simulink model "Prado23210715YP4"  (R2023a)
settings: Solver=VariableStepAuto  StartTime=0.0  StopTime=10.0  MaxStep=1E-3  RelTol=1e-3
libraries: fl_lib x14, nesl_utility x6, slpidlib x1
settings Model: Creator=adrib  LastModifiedBy=IT
settings DataIOCC: SaveFormat=Array  ReturnWorkspaceOutputs=off  TimeSaveName=t
settings DebuggingCC: AlgebraicLoopMsg=none  ArtificialAlgebraicLoopMsg=none  MaxConsecutiveZCsMsg=none  ModelReferenceExtraNoncontSigs=none  OperatingPointInterfaceChecksumMismatchMsg=none

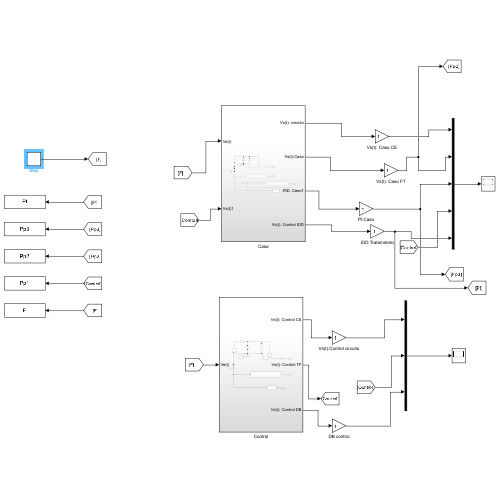
[thumbnail: Simulink's stored preview of the top-level diagram]
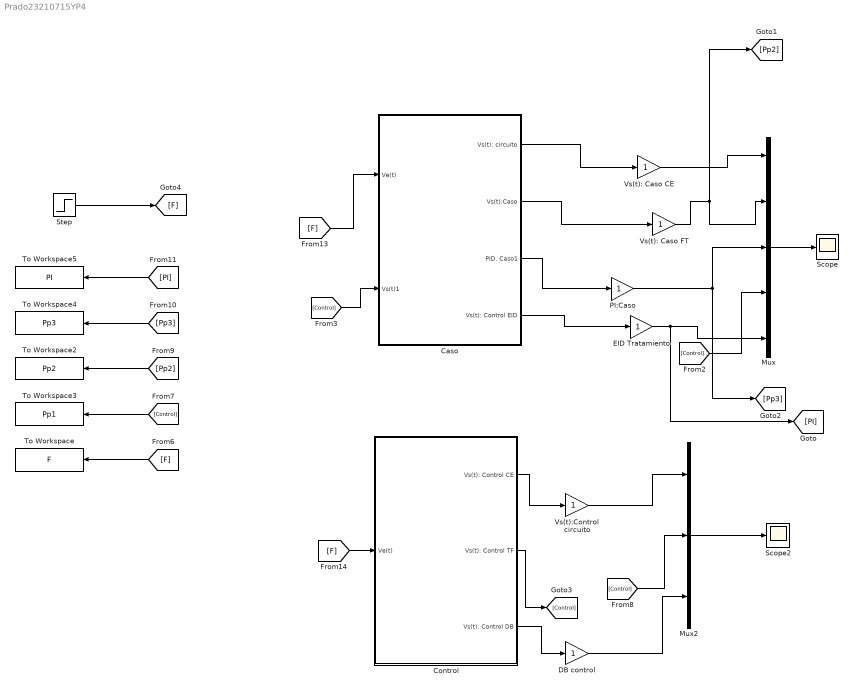
== system Prado23210715YP4 ==
  Caso : Subsystem
  Control : Subsystem
  DB control : Gain
  EID Tratamiento : Gain
  Mux : Mux  Inputs=5
  Mux2 : Mux  Inputs=3
  PI:Caso : Gain
  Scope : Scope
  Scope2 : Scope
  Step : Step  Time=0  SampleTime=0
  To Workspace : ToWorkspace  VariableName=F  SampleTime=-1
  To Workspace2 : ToWorkspace  VariableName=Pp2  SampleTime=-1
  To Workspace3 : ToWorkspace  VariableName=Pp1  SampleTime=-1
  To Workspace4 : ToWorkspace  VariableName=Pp3  SampleTime=-1
  To Workspace5 : ToWorkspace  VariableName=PI  SampleTime=-1
  Vs(t): Caso CE : Gain
  Vs(t): Caso FT : Gain
  Vs(t):Control circuito : Gain
  wires:
  Mux/1 -> Scope/1
  Mux2/1 -> Scope2/1
  [F] -> To Workspace/1
  [Control] -> To Workspace3/1
  [Pp2] -> To Workspace2/1
  [Pp3] -> To Workspace4/1
  [PI] -> To Workspace5/1
  [F] -> Control/1(Ve(t))
  Step/1 -> [F]
  Caso/1(Vs(t): circuito) -> Vs(t): Caso CE/1
  Vs(t): Caso FT/1 -> [Pp2], Mux/2
  [F] -> Caso/1(Ve(t))
  Caso/2(Vs(t):Caso) -> Vs(t): Caso FT/1
  Caso/3(PID. Caso1) -> PI:Caso/1
  [Control] -> Mux/4
  [Control] -> Caso/2(Vs(t)1)
  Control/2(Vs(t): Control TF) -> [Control]
  [Control] -> Mux2/2
  Control/1(Vs(t): Control CE) -> Vs(t):Control circuito/1
  Vs(t):Control circuito/1 -> Mux2/1
  Caso/4(Vs(t): Control EID) -> EID Tratamiento/1
  EID Tratamiento/1 -> [PI], Mux/5
  Control/3(Vs(t): Control DB) -> DB control/1
  DB control/1 -> Mux2/3
  Vs(t): Caso CE/1 -> Mux/1
  PI:Caso/1 -> [Pp3], Mux/3

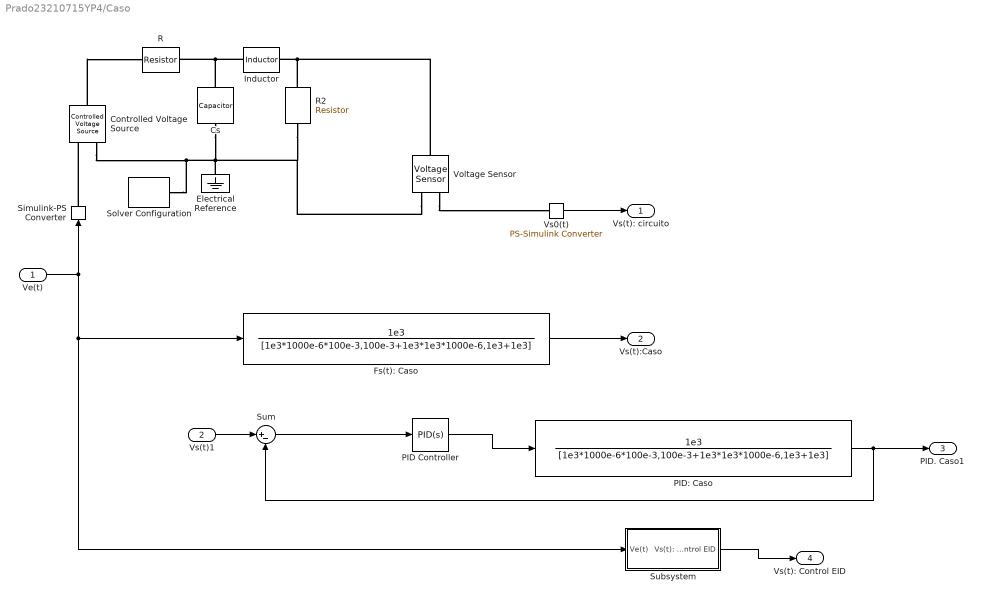
== system Prado23210715YP4/Caso ==
  Ve(t) : Inport
  Vs(t)1 : Inport  Port=2
  Controlled Voltage Source : fl_lib/Electrical/Electrical Sources/Controlled Voltage Source
  Cs : fl_lib/Electrical/Electrical Elements/Capacitor  c=1000e-6 F  r=1e-6 Ohm  g=0 1/Ohm  i_specify=off  i_priority=None  i=0 A  i_nominal_specify=off  i_nominal_unit=A  i_nominal_value=1  v_specify=off  v_priority=None  v=0 V  v_nominal_specify=off  v_nominal_unit=V  v_nominal_value=1  vc_specify=off  vc_priority=High  vc=0 V  vc_nominal_specify=off  vc_nominal_unit=V  vc_nominal_value=1
  Electrical Reference : fl_lib/Electrical/Electrical Elements/Electrical Reference
  Fs(t): Caso : TransferFcn  Numerator=[1e3]  Denominator=[1e3*1000e-6*100e-3,100e-3+1e3*1e3*1000e-6,1e3+1e3]
  Inductor : fl_lib/Electrical/Electrical Elements/Inductor  l=100e-3 H  r=0 Ohm  g=1e-9 1/Ohm  i_specify=off  i_priority=None  i=0 A  i_nominal_specify=off  i_nominal_unit=A  i_nominal_value=1  v_specify=off  v_priority=None  v=0 V  v_nominal_specify=off  v_nominal_unit=V  v_nominal_value=1  i_L_specify=off  i_L_priority=High  i_L=0 A  i_L_nominal_specify=off  i_L_nominal_unit=A  i_L_nominal_value=1
  PID Controller : slpidlib/PID Controller  Controller=PID  Form=Parallel  TimeDomain=Continuous-time  UseExternalTs=off  SampleTime=-1  IntegratorMethod=Forward Euler  FilterMethod=Forward Euler  ControllerParametersSource=internal  P=1315.6500509428  I=314901.771136491  UseKiTs=off  D=0.310353252867865  N=7592.76369465997  UseFilter=on  TunerSelectOption=Transfer Function Based (PID Tuner App)  InitialConditionSource=internal  InitialConditionForIntegrator=0  InitialConditionForFilter=0  DifferentiatorICPrevScaledInput=0  ExternalReset=none  TrackingMode=off  Kt=1  LimitOutput=off  SatLimitsSource=internal  UpperSaturationLimit=inf  LowerSaturationLimit=-inf  LinearizeAsGain=on  AntiWindupMode=none  Kb=1  LimitIntegrator=off  UpperIntegratorSaturationLimit=inf  LowerIntegratorSaturationLimit=-inf  POutMin=[]  POutMax=[]  IOutMin=[]  IOutMax=[]  DOutMin=[]  DOutMax=[]  NOutMin=[]  NOutMax=[]  SumOutMin=[]  SumOutMax=[]  SaturationOutMin=[]  SaturationOutMax=[]  PParamMin=[]  PParamMax=[]  IParamMin=[]  IParamMax=[]  DParamMin=[]  DParamMax=[]  NParamMin=[]  NParamMax=[]  KbParamMin=[]  KbParamMax=[]  KtParamMin=[]  KtParamMax=[]  KbOutMin=[]  KbOutMax=[]  KtOutMin=[]  KtOutMax=[]  IntegratorOutMin=[]  IntegratorOutMax=[]  FilterOutMin=[]  FilterOutMax=[]  SumI1OutMin=[]  SumI1OutMax=[]  SumI2OutMin=[]  SumI2OutMax=[]  SumI3OutMin=[]  SumI3OutMax=[]  SumI4OutMin=[]  SumI4OutMax=[]  SumDOutMin=[]  SumDOutMax=[]  DifferentiatorOutMin=[]  DifferentiatorOutMax=[]  FilterDiffOutCoefMin=[]  FilterDiffOutCoefMax=[]  ReciprocalOutMin=[]  ReciprocalOutMax=[]  SumDenOutMin=[]  SumDenOutMax=[]  SumNumOutMin=[]  SumNumOutMax=[]  DivideOutMin=[]  DivideOutMax=[]  UdiffTsProdOutMin=[]  UdiffTsProdOutMax=[]  NTsProdOutMin=[]  NTsProdOutMax=[]  UintegralTsProdOutMin=[]  UintegralTsProdOutMax=[]  UngainTsProdOutMin=[]  UngainTsProdOutMax=[]  ClampingZeroOutDataTypeStr=Inherit: Inherit via back propagation  ClampingZeroOutMin=[]  ClampingZeroOutMax=[]  FilterDenConstantOutDataTypeStr=Inherit: Inherit via back propagation  FilterDenConstantOutMin=[]  FilterDenConstantOutMax=[]  PCopyOutDataTypeStr=Inherit: Inherit via back propagation  PCopyOutMin=[]  PCopyOutMax=[]  NCopyOutDataTypeStr=Inherit: Inherit via back propagation  NCopyOutMin=[]  NCopyOutMax=[]  IntegratorContinuousStateAttributes=''  IntegratorStateMustResolveToSignalObject=off  IntegratorRTWStateStorageClass=Auto  FilterContinuousStateAttributes=''  FilterStateMustResolveToSignalObject=off  FilterRTWStateStorageClass=Auto  ParallelPVariant=InternalParameters  IdealPVariant=Disabled  IVariant=InternalParameters  DVariant=InternalParameters  IntegratorVariant=Continuous  SatVariant=Disabled  AWVariant=Passthrough  PCopyVariant=Disabled  TRVariant=Disabled  FdbkBlocksVariant=Forward  IdealPFdbkVariant=Disabled  SatFdbkVariant=Disabled  DerivativeFilterVariant=ContFilter  NVariant=InternalParameters  NCopyVariant=Disabled  FilterICVariant=InternalICsFilter  IntegratorICVariant=InternalICs  ExternalResetVariant=Disabled  TRSumVariant=Passthrough  SumFdbkVariant=Disabled  SumVariant=Sum_PID  TsampFilterVariant=InternalTs  TsampNgainVariant=Passthrough  TsampIntegralVariant=Disabled_SignalSpec  ExternalSaturationOutDataTypeStr=Inherit: Same as second input
  PID: Caso : TransferFcn  Numerator=[1e3]  Denominator=[1e3*1000e-6*100e-3,100e-3+1e3*1e3*1000e-6,1e3+1e3]
  R : fl_lib/Electrical/Electrical Elements/Resistor  R=1 kOhm  i_specify=off  i_priority=None  i=0 A  i_nominal_specify=off  i_nominal_unit=A  i_nominal_value=1  v_specify=off  v_priority=None  v=0 V  v_nominal_specify=off  v_nominal_unit=V  v_nominal_value=1
  R2 : fl_lib/Electrical/Electrical Elements/Resistor  R=1 kOhm  i_specify=off  i_priority=None  i=0 A  i_nominal_specify=off  i_nominal_unit=A  i_nominal_value=1  v_specify=off  v_priority=None  v=0 V  v_nominal_specify=off  v_nominal_unit=V  v_nominal_value=1
  Simulink-PS Converter : nesl_utility/Simulink-PS Converter  PhysicalDomain=network_engine_domain  SubClassName=ps_input  LeftPortType=input  RightPortType=output  PseudoPeriodic=off  Frequencies=[]  NoiseDistribution=none  NoiseParameters=[]  Unit=1  AffineConversion=off  FilteringAndDerivatives=provide  SimscapeFilterOrder=1  InputFilterTimeConstant=0.001  UdotUserProvided=0
  Solver Configuration : nesl_utility/Solver Configuration  PhysicalDomain=network_engine_domain  SubClassName=solver  LeftPortType=input  RightPortType=generic  Tones=[]  Harmonics=[]  SimulateNoise=off  Profile=off  UseLocalSampling=off  EnableSwitchedLinearOptims=on  FrequencyDomain=off  UseCCode=off  RelTol=0.001  AbsTol=0.001  MinStep=1e-09  ToWorkspace=off  RevertToSquareIcSolve=off  NumHomotopyIterations=100  PhasorMode=off  PhasorModeNumHarmonics=1  ConsistencySolver=NEWTON_XTOL_AFTER_FTOL  IndexReductionMethod=DerivativeReplacement  DoDC=off  ResidualTolerance=1e-09  ConsistencyTolSource=GLOBAL  ConsistencyAbsTol=0.001  ConsistencyRelTol=0.001  ConsistencyTolFactor=0.001  UseLocalSolver=off  LocalSolverChoice=NE_BACKWARD_EULER_ADVANCER  ResolveIndetEquations=on  FunctionEvalNumThread=1  LocalSolverSampleTime=0.001  DoFixedCost=off  MaxNonlinIter=3  MaxModeIter=2  ComputeImpulses=off  ImpulseIterations=2  LinearAlgebra=auto  LinearAlgebraNumThread=0  EquationFormulation=NE_TIME_EF  DelaysMemoryBudget=1024  AutomaticFiltering=on  FilteringTimeConstant=0.001  PartitionStorageMethod=AS_NEEDED  PartitionMemoryBudget=1024  PartitionMethod=ROBUST
  Subsystem : Subsystem
  Sum : Sum  Inputs=|+-
  Voltage Sensor : fl_lib/Electrical/Electrical Sensors/Voltage Sensor
  Vs0(t) : nesl_utility/PS-Simulink Converter  PhysicalDomain=network_engine_domain  SubClassName=ps_output  LeftPortType=input  RightPortType=output  PseudoPeriodic=off  Frequencies=[]  VectorFormat=1-D array  Unit=inherit  AffineConversion=off
  Vs(t): circuito : Outport
  Vs(t):Caso : Outport  Port=2
  PID. Caso1 : Outport  Port=3
  Vs(t): Control EID : Outport  Port=4
  wires:
  Fs(t): Caso/1 -> Vs(t):Caso/1
  Vs0(t)/1 -> Vs(t): circuito/1
  Ve(t)/1 -> Simulink-PS Converter/1, Subsystem/1(Ve(t)), Fs(t): Caso/1
  Sum/1 -> PID Controller/1
  PID: Caso/1 -> Sum/2, PID. Caso1/1
  PID Controller/1 -> PID: Caso/1
  Vs(t)1/1 -> Sum/1
  Subsystem/1(Vs(t): Control EID) -> Vs(t): Control EID/1
  connections:
  Controlled Voltage Source/RConn2 -- R2/LConn1 -- Voltage Sensor/RConn2 -- Cs/LConn1 -- Electrical Reference/LConn1 -- Solver Configuration/RConn1
  Voltage Sensor/RConn1 -- Vs0(t)/LConn1
  Simulink-PS Converter/RConn1 -- Controlled Voltage Source/RConn1
  Controlled Voltage Source/LConn1 -- R/RConn1
  Inductor/LConn1 -- Cs/RConn1 -- R/LConn1
  Voltage Sensor/LConn1 -- R2/RConn1 -- Inductor/RConn1

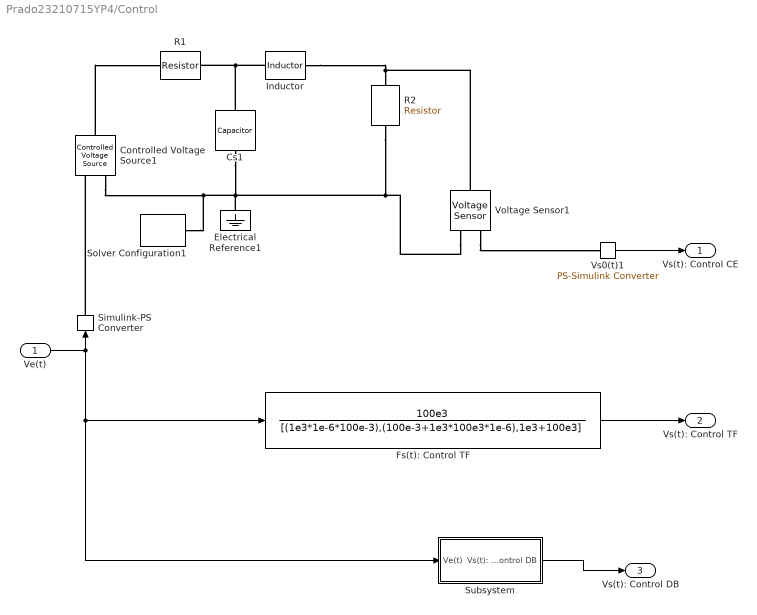
== system Prado23210715YP4/Control ==
  Ve(t) : Inport
  Controlled Voltage Source1 : fl_lib/Electrical/Electrical Sources/Controlled Voltage Source
  Cs1 : fl_lib/Electrical/Electrical Elements/Capacitor  c=1e-6 F  r=1e-6 Ohm  g=0 1/Ohm  i_specify=off  i_priority=None  i=0 A  i_nominal_specify=off  i_nominal_unit=A  i_nominal_value=1  v_specify=off  v_priority=None  v=0 V  v_nominal_specify=off  v_nominal_unit=V  v_nominal_value=1  vc_specify=off  vc_priority=High  vc=0 V  vc_nominal_specify=off  vc_nominal_unit=V  vc_nominal_value=1
  Electrical Reference1 : fl_lib/Electrical/Electrical Elements/Electrical Reference
  Fs(t): Control TF : TransferFcn  Numerator=[100e3]  Denominator=[(1e3*1e-6*100e-3),(100e-3+1e3*100e3*1e-6),1e3+100e3]
  Inductor : fl_lib/Electrical/Electrical Elements/Inductor  l=100e-3 H  r=0 Ohm  g=1e-9 1/Ohm  i_specify=off  i_priority=None  i=0 A  i_nominal_specify=off  i_nominal_unit=A  i_nominal_value=1  v_specify=off  v_priority=None  v=0 V  v_nominal_specify=off  v_nominal_unit=V  v_nominal_value=1  i_L_specify=off  i_L_priority=High  i_L=0 A  i_L_nominal_specify=off  i_L_nominal_unit=A  i_L_nominal_value=1
  R1 : fl_lib/Electrical/Electrical Elements/Resistor  R=1 kOhm  i_specify=off  i_priority=None  i=0 A  i_nominal_specify=off  i_nominal_unit=A  i_nominal_value=1  v_specify=off  v_priority=None  v=0 V  v_nominal_specify=off  v_nominal_unit=V  v_nominal_value=1
  R2 : fl_lib/Electrical/Electrical Elements/Resistor  R=100 kOhm  i_specify=off  i_priority=None  i=0 A  i_nominal_specify=off  i_nominal_unit=A  i_nominal_value=1  v_specify=off  v_priority=None  v=0 V  v_nominal_specify=off  v_nominal_unit=V  v_nominal_value=1
  Simulink-PS Converter : nesl_utility/Simulink-PS Converter  PhysicalDomain=network_engine_domain  SubClassName=ps_input  LeftPortType=input  RightPortType=output  PseudoPeriodic=off  Frequencies=[]  NoiseDistribution=none  NoiseParameters=[]  Unit=1  AffineConversion=off  FilteringAndDerivatives=provide  SimscapeFilterOrder=1  InputFilterTimeConstant=0.001  UdotUserProvided=0
  Solver Configuration1 : nesl_utility/Solver Configuration  PhysicalDomain=network_engine_domain  SubClassName=solver  LeftPortType=input  RightPortType=generic  Tones=[]  Harmonics=[]  SimulateNoise=off  Profile=off  UseLocalSampling=off  EnableSwitchedLinearOptims=on  FrequencyDomain=off  UseCCode=off  RelTol=0.001  AbsTol=0.001  MinStep=1e-09  ToWorkspace=off  RevertToSquareIcSolve=off  NumHomotopyIterations=100  PhasorMode=off  PhasorModeNumHarmonics=1  ConsistencySolver=NEWTON_XTOL_AFTER_FTOL  IndexReductionMethod=DerivativeReplacement  DoDC=off  ResidualTolerance=1e-09  ConsistencyTolSource=GLOBAL  ConsistencyAbsTol=0.001  ConsistencyRelTol=0.001  ConsistencyTolFactor=0.001  UseLocalSolver=off  LocalSolverChoice=NE_BACKWARD_EULER_ADVANCER  ResolveIndetEquations=on  FunctionEvalNumThread=1  LocalSolverSampleTime=0.001  DoFixedCost=off  MaxNonlinIter=3  MaxModeIter=2  ComputeImpulses=off  ImpulseIterations=2  LinearAlgebra=auto  LinearAlgebraNumThread=0  EquationFormulation=NE_TIME_EF  DelaysMemoryBudget=1024  AutomaticFiltering=on  FilteringTimeConstant=0.001  PartitionStorageMethod=AS_NEEDED  PartitionMemoryBudget=1024  PartitionMethod=ROBUST
  Subsystem : Subsystem
  Voltage Sensor1 : fl_lib/Electrical/Electrical Sensors/Voltage Sensor
  Vs0(t)1 : nesl_utility/PS-Simulink Converter  PhysicalDomain=network_engine_domain  SubClassName=ps_output  LeftPortType=input  RightPortType=output  PseudoPeriodic=off  Frequencies=[]  VectorFormat=1-D array  Unit=inherit  AffineConversion=off
  Vs(t): Control CE : Outport
  Vs(t): Control TF : Outport  Port=2
  Vs(t): Control DB : Outport  Port=3
  wires:
  Ve(t)/1 -> Subsystem/1(Ve(t)), Fs(t): Control TF/1, Simulink-PS Converter/1
  Vs0(t)1/1 -> Vs(t): Control CE/1
  Fs(t): Control TF/1 -> Vs(t): Control TF/1
  Subsystem/1(Vs(t): Control DB) -> Vs(t): Control DB/1
  connections:
  Controlled Voltage Source1/RConn2 -- R2/LConn1 -- Voltage Sensor1/RConn2 -- Cs1/RConn1 -- Electrical Reference1/LConn1 -- Solver Configuration1/RConn1
  Controlled Voltage Source1/LConn1 -- R1/RConn1
  Voltage Sensor1/RConn1 -- Vs0(t)1/LConn1
  Simulink-PS Converter/RConn1 -- Controlled Voltage Source1/RConn1
  Cs1/LConn1 -- R1/LConn1 -- Inductor/LConn1
  Inductor/RConn1 -- Voltage Sensor1/LConn1 -- R2/RConn1

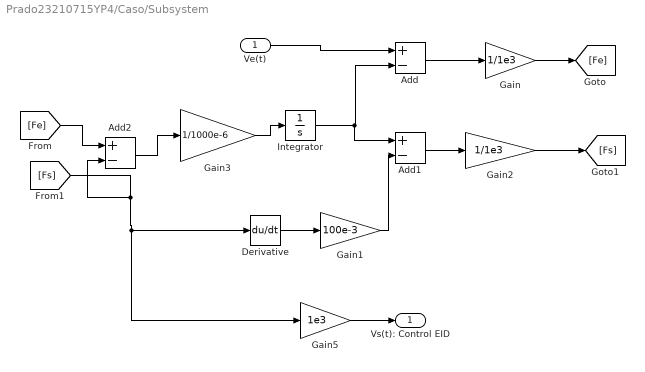
== system Prado23210715YP4/Caso/Subsystem ==
  Ve(t) : Inport
  Add : Sum  Inputs=+-
  Add1 : Sum  Inputs=+-
  Add2 : Sum  Inputs=+-
  Derivative : Derivative
  Gain : Gain  Gain=1/1e3
  Gain1 : Gain  Gain=100e-3
  Gain2 : Gain  Gain=1/1e3
  Gain3 : Gain  Gain=1/1000e-6
  Gain5 : Gain  Gain=1e3
  Integrator : Integrator
  Vs(t): Control EID : Outport
  wires:
  Ve(t)/1 -> Add/1
  Integrator/1 -> Add1/1, Add/2
  Add/1 -> Gain/1
  Add1/1 -> Gain2/1
  Derivative/1 -> Gain1/1
  Gain1/1 -> Add1/2
  Gain3/1 -> Integrator/1
  Add2/1 -> Gain3/1
  [Fe] -> Add2/1
  [Fs] -> Gain5/1, Derivative/1, Add2/2
  Gain5/1 -> Vs(t): Control EID/1
  Gain2/1 -> [Fs]
  Gain/1 -> [Fe]

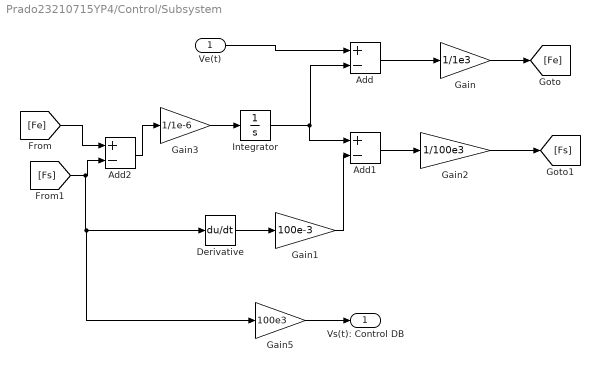
== system Prado23210715YP4/Control/Subsystem ==
  Ve(t) : Inport
  Add : Sum  Inputs=+-
  Add1 : Sum  Inputs=+-
  Add2 : Sum  Inputs=+-
  Derivative : Derivative
  Gain : Gain  Gain=1/1e3
  Gain1 : Gain  Gain=100e-3
  Gain2 : Gain  Gain=1/100e3
  Gain3 : Gain  Gain=1/1e-6
  Gain5 : Gain  Gain=100e3
  Integrator : Integrator
  Vs(t): Control DB : Outport
  wires:
  Ve(t)/1 -> Add/1
  Integrator/1 -> Add1/1, Add/2
  Add/1 -> Gain/1
  Add1/1 -> Gain2/1
  Derivative/1 -> Gain1/1
  Gain1/1 -> Add1/2
  Gain3/1 -> Integrator/1
  Add2/1 -> Gain3/1
  [Fe] -> Add2/1
  [Fs] -> Gain5/1, Derivative/1, Add2/2
  Gain5/1 -> Vs(t): Control DB/1
  Gain2/1 -> [Fs]
  Gain/1 -> [Fe]
